simulink model "mli_triphase"  (Simulink 7.4)
settings: Solver=FixedStepDiscrete  StartTime=0.0  StopTime=0.06  FixedStep=0.0001  RelTol=1e-3
undefined symbols (not defined in the file or in its folder): DiscIntNeverNeededParam
libraries: dsPICdrivers x4
settings Model: Creator=Safano  LastModifiedBy=ELMAY
settings OptimizationCC: OptimizeModelRefInitCode=on  LifeSpan=1
settings HardwareCC: ProdBitPerInt=16  ProdEndianess=LittleEndian  ProdWordSize=16  ProdHWDeviceType=16-bit Generic
settings RTWCC: SystemTargetFile=dspic.tlc  MakeCommand=make_CreateMPLAB  TemplateMakefile=dspic_pic30_gcc.tmf  PostCodeGenCommand=dsPIC_Compile()  Description=Embedded Target for Microchip dsPIC (real-time)  ProcessScript=dspic_make_rtw_hook
settings CodeAppCC: IgnoreCustomStorageClasses=off
settings STFCustomTargetCC: IncludeMdlTerminateFcn=off  CombineOutputUpdateFcns=on  SuppressErrorStatus=on  ERTCustomFileBanners=on  SupportContinuousTime=off  SupportNonInlinedSFcns=off  SystemTargetFile=dspic.tlc
settings ERTTargetCC: MultiwordLength=2048  ParMdlRefBuildCompliant=off  CompOptLevelCompliant=off  IncludeMdlTerminateFcn=off  SuppressErrorStatus=on  ERTFirstTimeCompliant=off  ModelStepFunctionPrototypeControlCompliant=off  CPPClassGenCompliant=off  ExtModeMexFile=ext_serial_win32_comm  InlinedParameterPlacement=NonHierarchical  ERTSrcFileBannerTemplate=dsPIC_code_template.cgt  ERTHdrFileBannerTemplate=dsPIC_code_template.cgt  ERTDataSrcFileTemplate=dsPIC_code_template.cgt  ERTDataHdrFileTemplate=dsPIC_code_template.cgt  ERTCustomFileTemplate=dsPIC_main.tlc  ConvertIfToSwitch=off
settings CustomProperty: DataType=string  Value=D:\PROGRA~1\MATLAB\R2009b\bin\win32\gmake

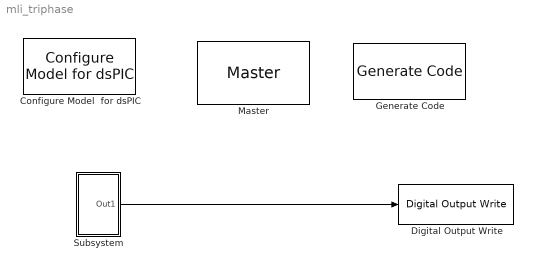
== system mli_triphase ==
  Configure Model  for dsPIC : dsPICdrivers/Simulink Configuration/Configure Model  for dsPIC
  Digital Output Write : dsPICdrivers/Digital I//O/Digital Output Write  Tag=dsPIC_Digital_Output  Priority=5  PORT=B  Pin=[0]  Simultaneous=off  OrderingInOutPopup=None
  Generate Code : dsPICdrivers/Simulink Configuration/Generate Code
  Master : dsPICdrivers/Master  Tag=dsPIC_MASTER  Priority=1  TimeStepType=Timer1  picType=30f4011  fcy=29.44e6  Quartz_33f=5e6  PLLActive_33f=off  fcyDesired_33f=0  tmr1="[1  2943  0]"  tmr1Info="Time Step : 0.0001  ;   Error : 0%  PR1=2943"  tmr2345="[0  0  0  0]"  tmr2345cfg=[-1 -1 -1 -1]  IOautoConf=on  typePort="[ 0   0   0   0   0   0   0   0   0   0   0   0   0   0   0   0  10   0   0   0   0   0   0   0   0   0   0   0   0   0   0   0   0   0   0   0   0   0   0   0   0   0   0   0   0   0   0   0   0   0   0   0   0   0   0   0   0   0   0   0   0   0   0   0   0   0   0   0   0   0   0   0   0   0   0   0   0   0   0   0   0   0   0   0   0   0   0   0   0   0   0   0   0   0   0   0   0   0   0   0   0   0   0   0   0   0   0   0   0   0   0   0 ]"  TRIS="[ 65535  65534  65535  65535  65535  65535  65535 ]"  ADPCFG=1  MasterBusyPort=None  MasterOverloadPort=None  FOSC=XT_PLL16  ClockSwitchMonitor=Both disabled  TempProtection_33f=TEMP_ON  FPBOR=PBOR_OFF  PWRT=PWRT_OFF  MCLR=MCLR_DIS  ICD=ICS_PGD1  JTAGEN=JTAGEN_OFF  PowerSave=off  OverrideFcy=off  NewFcy=1e6  PR2345="[65535  65535  65535  65535]"
  Subsystem : Subsystem
  wires:
  Subsystem/1(Out1) -> Digital Output Write/1

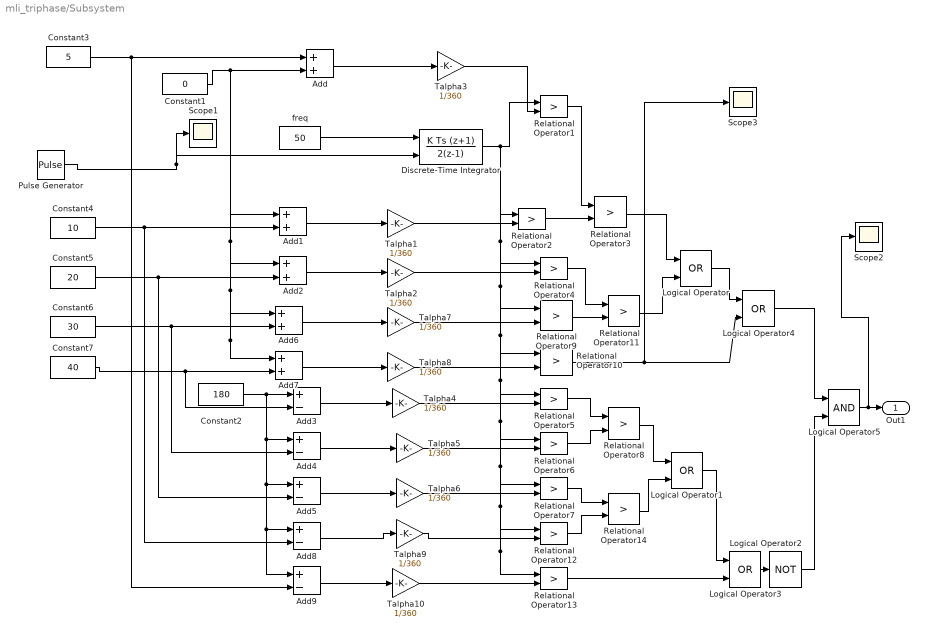
== system mli_triphase/Subsystem ==
  Add{,1..2,6..7} (5 alike) : Sum  OutDataType=fixdt(1, 16)  OutScaling=2^-10
  Add{3..5,8..9} (5 alike) : Sum  Inputs=+-  OutDataType=fixdt(1, 16)  OutScaling=2^-10
  Constant1 : Constant  Value=0  OutDataType=fixdt(1, 16)  OutScaling=2^0
  Constant2 : Constant  Value=180  OutDataType=fixdt(1, 16)  OutScaling=2^0
  Constant3 : Constant  Value=5  OutDataType=fixdt(1, 16)  OutScaling=2^0
  Constant4 : Constant  Value=10  OutDataType=fixdt(1, 16)  OutScaling=2^0
  Constant5 : Constant  Value=20  OutDataType=fixdt(1, 16)  OutScaling=2^0
  Constant6 : Constant  Value=30  OutDataType=fixdt(1, 16)  OutScaling=2^0
  Constant7 : Constant  Value=40  OutDataType=fixdt(1, 16)  OutScaling=2^0
  Discrete-Time Integrator : DiscreteIntegrator  IntegratorMethod=Integration: Trapezoidal  ExternalReset=rising  InitialConditionMode=State only (most efficient)  SampleTime=-1  OutDataType=sfix(16)  OutScaling=2^0  ICPrevOutput=DiscIntNeverNeededParam  ICPrevScaledInput=DiscIntNeverNeededParam
  Logical Operator{,1,3..4} (4 alike) : Logic  Operator=OR  AllPortsSameDT=off  OutDataTypeMode=boolean  LogicDataType=fixdt(0, 8)  OutDataTypeStr=boolean
  Logical Operator2 : Logic  Operator=NOT  AllPortsSameDT=off  OutDataTypeMode=boolean  LogicDataType=fixdt(0, 8)  OutDataTypeStr=boolean
  Logical Operator5 : Logic  AllPortsSameDT=off  OutDataTypeMode=boolean  LogicDataType=fixdt(0, 8)  OutDataTypeStr=boolean
  Pulse Generator : DiscretePulseGenerator  PulseType=Time based  Amplitude=1  Period=0.02  PulseWidth=50  PhaseDelay=0  SampleTime=1
  Relational Operator{1..14} (14 alike) : RelationalOperator  Operator=>  InputSameDT=on
  Scope1 : Scope
      settings: YMin=-1  YMax=1  SaveName=ScopeData2
  Scope2 : Scope
  Scope3 : Scope
  Talpha{1..10} (10 alike) : Gain  Gain=1/360  ParameterDataType=sfix(16)  ParameterScaling=2^0  OutDataType=sfix(16)  OutScaling=2^0  SaturateOnIntegerOverflow=on  OutDataTypeStr=Inherit: Same as input  ParamDataTypeStr=Inherit: Same as input
  freq : Constant  Value=50  OutDataType=sfix(16)  OutScaling=2^0  SampleTime=0.0001
  Out1 : Outport
  wires:
  Add9/1 -> Talpha10/1
  Talpha10/1 -> Relational Operator13/2
  Relational Operator13/1 -> Logical Operator3/2
  Logical Operator2/1 -> Logical Operator5/2
  Logical Operator4/1 -> Logical Operator5/1
  Logical Operator3/1 -> Logical Operator2/1
  Logical Operator1/1 -> Logical Operator3/1
  Relational Operator14/1 -> Logical Operator1/2
  Relational Operator7/1 -> Relational Operator14/1
  Relational Operator12/1 -> Relational Operator14/2
  Talpha9/1 -> Relational Operator12/2
  Add8/1 -> Talpha9/1
  Relational Operator10/1 -> Logical Operator4/2, Scope3/1
  Relational Operator11/1 -> Logical Operator/2
  Relational Operator9/1 -> Relational Operator11/2
  Talpha8/1 -> Relational Operator10/2
  Talpha7/1 -> Relational Operator9/2
  Add7/1 -> Talpha8/1
  Add6/1 -> Talpha7/1
  Constant7/1 -> Add7/2, Add3/2
  Constant6/1 -> Add6/2, Add4/2
  Constant2/1 -> Add3/1, Add4/1, Add5/1, Add8/1, Add9/1
  Add4/1 -> Talpha5/1
  Add5/1 -> Talpha6/1
  Constant5/1 -> Add2/2, Add5/2
  Constant4/1 -> Add1/2, Add8/2
  Add1/1 -> Talpha1/1
  Constant1/1 -> Add/2, Add1/1, Add2/1, Add6/1, Add7/1
  Constant3/1 -> Add/1, Add9/2
  Add/1 -> Talpha3/1
  Relational Operator8/1 -> Logical Operator1/1
  Relational Operator6/1 -> Relational Operator8/2
  Relational Operator5/1 -> Relational Operator8/1
  Talpha6/1 -> Relational Operator7/2
  Talpha5/1 -> Relational Operator6/2
  Add3/1 -> Talpha4/1
  Talpha4/1 -> Relational Operator5/2
  Relational Operator2/1 -> Relational Operator3/2
  Relational Operator3/1 -> Logical Operator/1
  Logical Operator/1 -> Logical Operator4/1
  Relational Operator4/1 -> Relational Operator11/1
  Add2/1 -> Talpha2/1
  Talpha2/1 -> Relational Operator4/2
  Pulse Generator/1 -> Scope1/1, Discrete-Time Integrator/2
  Talpha1/1 -> Relational Operator2/2
  freq/1 -> Discrete-Time Integrator/1
  Talpha3/1 -> Relational Operator1/2
  Discrete-Time Integrator/1 -> Relational Operator2/1, Relational Operator4/1, Relational Operator9/1, Relational Operator5/1, Relational Operator6/1, Relational Operator12/1, Relational Operator13/1, Relational Operator7/1, Relational Operator10/1, Relational Operator1/1
  Relational Operator1/1 -> Relational Operator3/1
  Logical Operator5/1 -> Out1/1, Scope2/1
